simulink library "TurnLightActLib"  (R2020b)
settings: Solver=VariableStepAuto  StartTime=0.0  StopTime=10.0  RelTol=1e-3
settings Model: Creator=Wangjianwen  LastModifiedBy=Wangjianwen

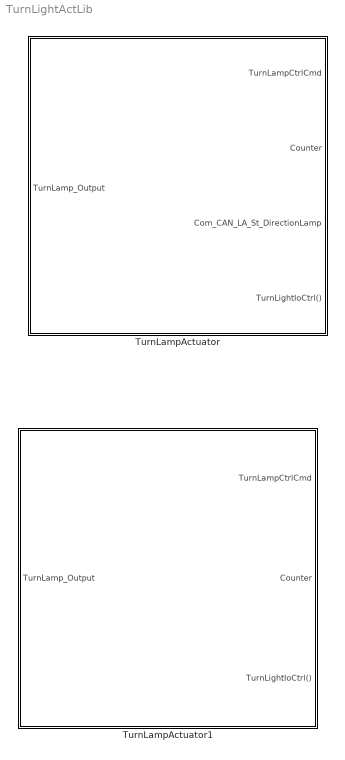
== system TurnLightActLib ==
  TurnLampActuator : Stateflow chart  TreatAsAtomicUnit=on
  TurnLampActuator1 : Stateflow chart  TreatAsAtomicUnit=on

== stateflow chart TurnLightActLib/TurnLampActuator1 ==
  state OFF
    en:
    TurnLampCtrlCmd = 0;
    TurnLightIoCtrl
  state Normal
    state OFF
      en:
      TurnLampCtrlCmd = 0;
      TurnLightIoCtrl
    state ON
      en:
      TurnLampCtrlCmd = 1;
      TurnLightIoCtrl
      ex:
      Counter = Counter+1;
    (default) -> Normal.OFF
    Normal.OFF -> Normal.ON : [after(40,tick)]
    Normal.ON -> Normal.OFF : [after(40,tick)]
  state Double
    state OFF
      en:
      TurnLampCtrlCmd = 0;
      TurnLightIoCtrl
    state ON
      en:
      TurnLampCtrlCmd =1;
      TurnLightIoCtrl
    (default) -> Double.OFF
    Double.OFF -> Double.ON : [after(20,tick)]
    Double.ON -> Double.OFF : [after(20,tick)]
  (default) -> OFF
  OFF -> Normal [order 1] : [TurnLamp_Output ==TLOUT_NORMAL_ON...
      | || TurnLamp_Output == TLOUT_SHORT_ON]{Counter = 0}
  Normal -> OFF [order 1] : [TurnLamp_Output ==TLOUT_SHORT_ON...
      | &&Counter == 3 ]
  Normal -> OFF [order 2] : [TurnLamp_Output ==TLOUT_OFF ]
  OFF -> Double [order 2] : [TurnLamp_Output == TLOUT_DOUBLE_ON]
  Double -> OFF : [TurnLamp_Output ==TLOUT_OFF ]
  data: TurnLamp_Output input; TurnLampCtrlCmd output uint8 =0; Counter output uint8 =0; TLOUT_OFF constant uint8 =0; TLOUT_NORMAL_ON constant uint8 =1; TLOUT_SHORT_ON constant uint8 =2; TLOUT_DOUBLE_ON constant uint8 =3
  events: TurnLightIoCtrl output FUNCTION_CALL_EVENT

== stateflow chart TurnLightActLib/TurnLampActuator ==
  state OFF
    en:
    Com_CAN_LA_St_DirectionLamp  =0;
    TurnLampCtrlCmd = 0;
    TurnLightIoCtrl
  state Normal
    state OFF
      en:
      TurnLampCtrlCmd = 0;
      Com_CAN_LA_St_DirectionLamp = 0;
      TurnLightIoCtrl
    state ON
      en:
      TurnLampCtrlCmd = 1;
      Com_CAN_LA_St_DirectionLamp = 1;
      TurnLightIoCtrl
      ex:
      Counter = Counter+1;
    (default) -> Normal.OFF
    Normal.OFF -> Normal.ON : [after(40,tick)]
    Normal.ON -> Normal.OFF : [after(40,tick)]
  state Double
    state OFF
      en:
      TurnLampCtrlCmd = 0;
      Com_CAN_LA_St_DirectionLamp = 0;
      TurnLightIoCtrl
    state ON
      en:
      TurnLampCtrlCmd =1;
      Com_CAN_LA_St_DirectionLamp = 1;
      TurnLightIoCtrl
    (default) -> Double.OFF
    Double.OFF -> Double.ON : [after(20,tick)]
    Double.ON -> Double.OFF : [after(20,tick)]
  (default) -> OFF
  OFF -> Normal [order 1] : [TurnLamp_Output ==TLOUT_NORMAL_ON...
      | || TurnLamp_Output == TLOUT_SHORT_ON]{Counter = 0}
  Normal -> OFF [order 1] : [TurnLamp_Output ==TLOUT_SHORT_ON...
      | &&Counter == 3 ]
  Normal -> OFF [order 2] : [TurnLamp_Output ==TLOUT_OFF ]
  OFF -> Double [order 2] : [TurnLamp_Output == TLOUT_DOUBLE_ON]
  Double -> OFF : [TurnLamp_Output ==TLOUT_OFF ]
  data: TurnLamp_Output input; TurnLampCtrlCmd output uint8 =0; Counter output uint8 =0; TLOUT_OFF constant uint8 =0; TLOUT_NORMAL_ON constant uint8 =1; TLOUT_SHORT_ON constant uint8 =2; TLOUT_DOUBLE_ON constant uint8 =3; Com_CAN_LA_St_DirectionLamp output uint8 =0
  events: TurnLightIoCtrl output FUNCTION_CALL_EVENT
